simulink model "sfInsectExample"  (R2025b)
settings: Solver=VariableStepAuto  StartTime=0.0  StopTime=24  RelTol=1e-3
PreLoadFcn:
  | load('insect_sim_consts.mat')
  | load('raw_enviro_data.mat')
values from neighbouring files (symbols this model uses):
  cone_angle = 45    [generate_constants.m]
  cone_length = 30    [generate_constants.m]
  fast_vel = 9    [generate_constants.m]
  norm_vel = 6    [generate_constants.m]
  x_bound = [0 100]    [generate_constants.m]
  y_bound = [0 75]    [generate_constants.m]
libraries: simulink_extras x2
settings Model: Creator=The MathWorks, Inc.  LastModifiedBy=The MathWorks, Inc.
settings DataIOCC: ExternalInput=[raw_enviro_data(:,5), raw_enviro_data]  LoadExternalInput=on
settings OptimizationCC: ReuseModelBlockBuffer=off
settings DebuggingCC: UnconnectedInputMsg=warning  UnconnectedOutputMsg=warning  UnconnectedLineMsg=warning
settings ModelReferenceCC: EnableRefExpFcnMdlSchedulingChecks=on
settings RTWCC: GPUComputeCapability=3.5  DLArmComputeVersion=19.05

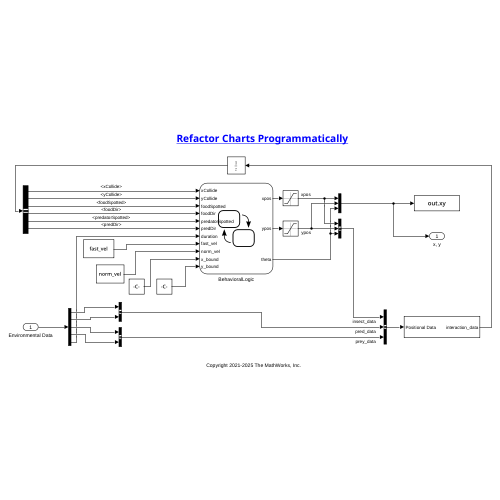
[thumbnail: Simulink's stored preview of the top-level diagram]
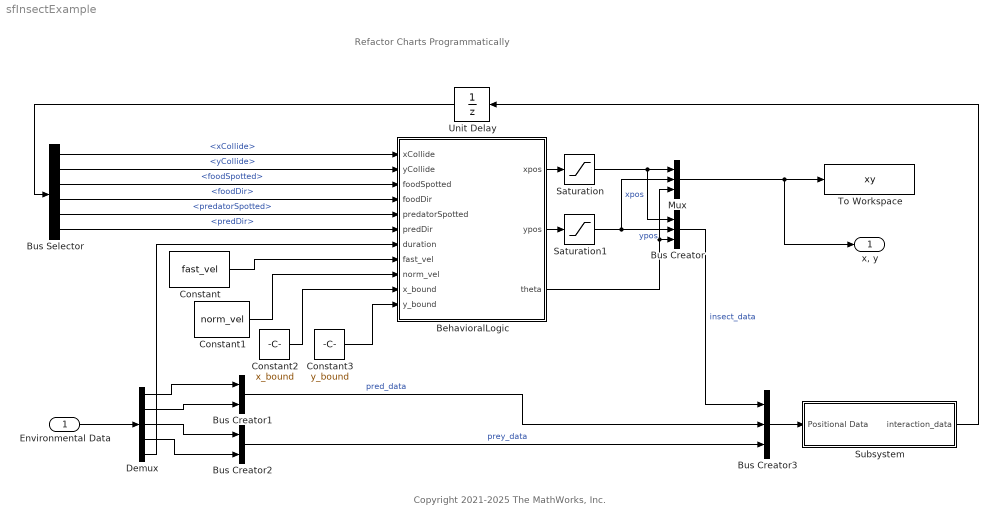
== system sfInsectExample ==
  note: Copyright 2021-2025 The MathWorks, Inc.
  note: Refactor Charts Programmatically
  Environmental Data : Inport
  BehavioralLogic : Stateflow chart  TreatAsAtomicUnit=on
  Bus Creator : BusCreator  Inputs=3
  Bus Creator1 : BusCreator  Inputs=2
  Bus Creator2 : BusCreator  Inputs=2
  Bus Creator3 : BusCreator  Inputs=3
  Bus Selector : BusSelector  OutputSignals=xCollide,yCollide,foodSpotted,foodDir,predatorSpotted,predDir
  Constant : Constant  Value=fast_vel
  Constant1 : Constant  Value=norm_vel
  Constant2 : Constant  Value=x_bound
  Constant3 : Constant  Value=y_bound
  Demux : Demux  Outputs=5
  Mux : Mux  Inputs=3
  Saturation : Saturate  UpperLimit=x_bound(2)  LowerLimit=x_bound(1)
  Saturation1 : Saturate  UpperLimit=y_bound(2)  LowerLimit=y_bound(1)
  Subsystem : Subsystem
  To Workspace : ToWorkspace  VariableName=xy  SampleTime=-1
  Unit Delay : UnitDelay  SampleTime=-1  HasFrameUpgradeWarning=on
  "x, y" : Outport
  wires:
  BehavioralLogic/3(theta) -> Mux/3, Bus Creator/3
  Environmental Data/1 -> Demux/1
  Demux/3 -> Bus Creator2/1
  Demux/4 -> Bus Creator2/2
  Bus Creator3/1 -> Subsystem/1(Positional Data)
  Bus Creator/1 -> Bus Creator3/1  "insect_data"
  Bus Creator1/1 -> Bus Creator3/2  "pred_data"
  Bus Creator2/1 -> Bus Creator3/3  "prey_data"
  Subsystem/1(interaction_data) -> Unit Delay/1
  Bus Selector/1 -> BehavioralLogic/1(xCollide)  "<xCollide>"
  Bus Selector/2 -> BehavioralLogic/2(yCollide)  "<yCollide>"
  Bus Selector/3 -> BehavioralLogic/3(foodSpotted)  "<foodSpotted>"
  Bus Selector/4 -> BehavioralLogic/4(foodDir)  "<foodDir>"
  Bus Selector/5 -> BehavioralLogic/5(predatorSpotted)  "<predatorSpotted>"
  Bus Selector/6 -> BehavioralLogic/6(predDir)  "<predDir>"
  Mux/1 -> To Workspace/1, "x, y"/1
  Demux/1 -> Bus Creator1/1
  Demux/2 -> Bus Creator1/2
  Demux/5 -> BehavioralLogic/7(duration)
  Constant/1 -> BehavioralLogic/8(fast_vel)
  Constant1/1 -> BehavioralLogic/9(norm_vel)
  Unit Delay/1 -> Bus Selector/1
  BehavioralLogic/1(xpos) -> Saturation/1
  Saturation/1 -> Mux/1, Bus Creator/1  "xpos"
  BehavioralLogic/2(ypos) -> Saturation1/1
  Saturation1/1 -> Mux/2, Bus Creator/2  "ypos"
  Constant2/1 -> BehavioralLogic/10(x_bound)
  Constant3/1 -> BehavioralLogic/11(y_bound)

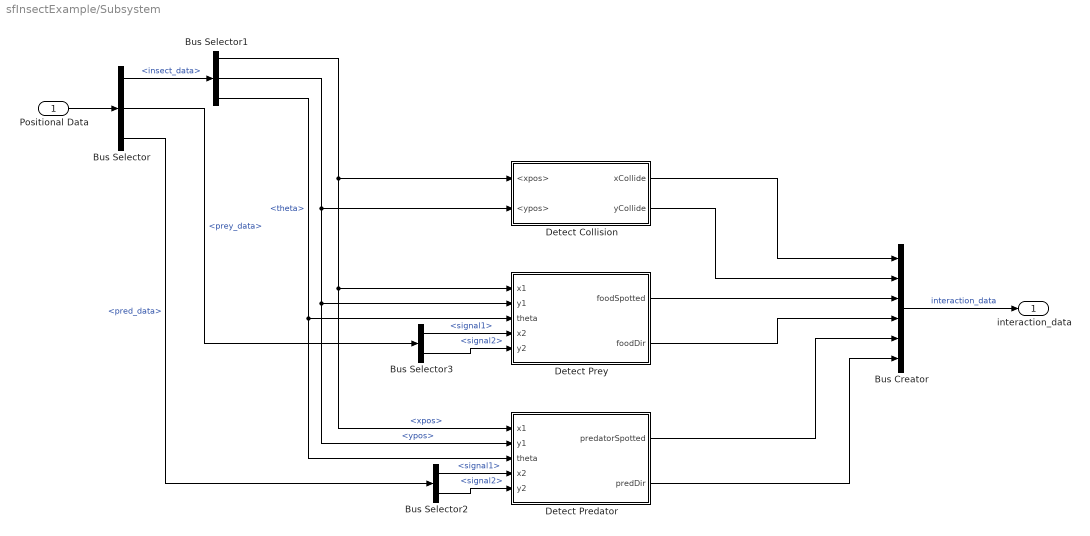
== system sfInsectExample/Subsystem ==
  Positional Data : Inport
  Bus Creator : BusCreator  Inputs=6
  Bus Selector : BusSelector  OutputSignals=insect_data,prey_data,pred_data
  Bus Selector1 : BusSelector  OutputSignals=xpos,ypos,theta
  Bus Selector2 : BusSelector  OutputSignals=signal1,signal2
  Bus Selector3 : BusSelector  OutputSignals=signal1,signal2
  Detect Collision : Subsystem
  "Detect Predator " : Subsystem
  Detect Prey : Subsystem
  interaction_data : Outport
  wires:
  Positional Data/1 -> Bus Selector/1
  Bus Selector/1 -> Bus Selector1/1  "<insect_data>"
  Bus Selector1/1 -> Detect Collision/1(<xpos>), Detect Prey/1(x1), "Detect Predator "/1(x1)  "<xpos>"
  Bus Selector1/2 -> Detect Collision/2(<ypos>), Detect Prey/2(y1), "Detect Predator "/2(y1)  "<ypos>"
  Bus Selector/3 -> Bus Selector2/1  "<pred_data>"
  Bus Selector2/1 -> "Detect Predator "/4(x2)  "<signal1>"
  Bus Selector2/2 -> "Detect Predator "/5(y2)  "<signal2>"
  Bus Selector1/3 -> Detect Prey/3(theta), "Detect Predator "/3(theta)  "<theta>"
  Bus Selector3/1 -> Detect Prey/4(x2)  "<signal1>"
  Bus Selector/2 -> Bus Selector3/1  "<prey_data>"
  Bus Selector3/2 -> Detect Prey/5(y2)  "<signal2>"
  Detect Collision/1(xCollide) -> Bus Creator/1
  Detect Collision/2(yCollide) -> Bus Creator/2
  Detect Prey/1(foodSpotted) -> Bus Creator/3
  Detect Prey/2(foodDir) -> Bus Creator/4
  "Detect Predator "/1(predatorSpotted) -> Bus Creator/5
  "Detect Predator "/2(predDir) -> Bus Creator/6
  Bus Creator/1 -> interaction_data/1  "interaction_data"

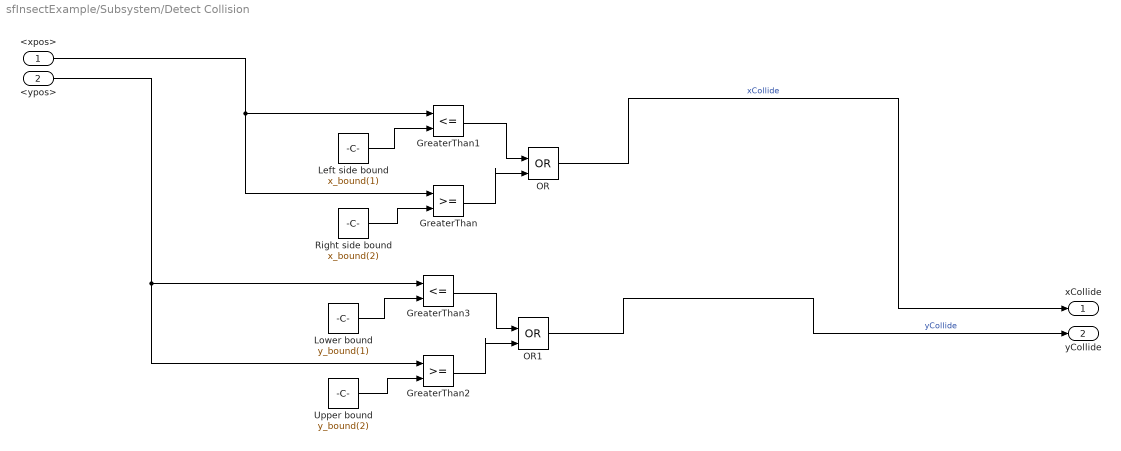
== system sfInsectExample/Subsystem/Detect Collision ==
  <xpos> : Inport
  <ypos> : Inport  Port=2
  GreaterThan : RelationalOperator  OutDataTypeStr=boolean  RndMeth=Simplest  InputSameDT=off
  GreaterThan1 : RelationalOperator  Operator=<=  OutDataTypeStr=boolean  RndMeth=Simplest  InputSameDT=off
  GreaterThan2 : RelationalOperator  OutDataTypeStr=boolean  RndMeth=Simplest  InputSameDT=off
  GreaterThan3 : RelationalOperator  Operator=<=  OutDataTypeStr=boolean  RndMeth=Simplest  InputSameDT=off
  Left side bound : Constant  Value=x_bound(1)
  Lower bound : Constant  Value=y_bound(1)
  OR : Logic  Operator=OR  IconShape=distinctive  AllPortsSameDT=off  OutDataTypeStr=boolean
  OR1 : Logic  Operator=OR  IconShape=distinctive  AllPortsSameDT=off  OutDataTypeStr=boolean
  Right side bound : Constant  Value=x_bound(2)
  Upper bound : Constant  Value=y_bound(2)
  xCollide : Outport
  yCollide : Outport  Port=2
  wires:
  GreaterThan2/1 -> OR1/2
  Upper bound/1 -> GreaterThan2/2
  GreaterThan1/1 -> OR/1
  Right side bound/1 -> GreaterThan/2
  Left side bound/1 -> GreaterThan1/2
  Lower bound/1 -> GreaterThan3/2
  <ypos>/1 -> GreaterThan3/1, GreaterThan2/1
  GreaterThan3/1 -> OR1/1
  <xpos>/1 -> GreaterThan1/1, GreaterThan/1
  GreaterThan/1 -> OR/2
  OR/1 -> xCollide/1  "xCollide"
  OR1/1 -> yCollide/1  "yCollide"

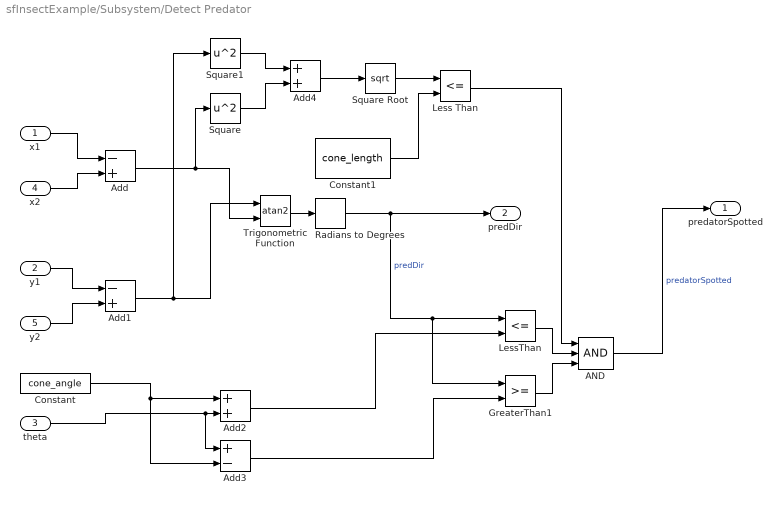
== system sfInsectExample/Subsystem/Detect Predator  ==
  x1 : Inport
  y1 : Inport  Port=2
  theta : Inport  Port=3
  x2 : Inport  Port=4
  y2 : Inport  Port=5
  AND : Logic  Inputs=3  IconShape=distinctive  AllPortsSameDT=off  OutDataTypeStr=boolean
  Add : Sum  Inputs=-+
  Add1 : Sum  Inputs=-+
  Add2 : Sum
  Add3 : Sum  Inputs=+-
  Add4 : Sum
  Constant : Constant  Value=cone_angle
  Constant1 : Constant  Value=cone_length
  GreaterThan1 : RelationalOperator  OutDataTypeStr=boolean  RndMeth=Simplest  InputSameDT=off
  Less Than : RelationalOperator  Operator=<=  OutDataTypeStr=boolean  RndMeth=Simplest  InputSameDT=off
  LessThan : RelationalOperator  Operator=<=  OutDataTypeStr=boolean  RndMeth=Simplest  InputSameDT=off
  Radians to Degrees : simulink_extras/Transformations/Radians to Degrees
  Square : Math  Operator=square
  Square Root : Sqrt
  Square1 : Math  Operator=square
  Trigonometric Function : Trigonometry  Operator=atan2
  predatorSpotted : Outport
  predDir : Outport  Port=2
  wires:
  x1/1 -> Add/1
  x2/1 -> Add/2
  y1/1 -> Add1/1
  y2/1 -> Add1/2
  Add1/1 -> Trigonometric Function/1, Square1/1
  Add/1 -> Square/1, Trigonometric Function/2
  Trigonometric Function/1 -> Radians to Degrees/1
  Radians to Degrees/1 -> predDir/1, GreaterThan1/1, LessThan/1  "predDir"
  theta/1 -> Add3/1, Add2/2
  Constant/1 -> Add3/2, Add2/1
  Add2/1 -> LessThan/2
  Add3/1 -> GreaterThan1/2
  LessThan/1 -> AND/2
  GreaterThan1/1 -> AND/3
  Square1/1 -> Add4/1
  Square/1 -> Add4/2
  Add4/1 -> Square Root/1
  Square Root/1 -> Less Than/1
  Constant1/1 -> Less Than/2
  Less Than/1 -> AND/1
  AND/1 -> predatorSpotted/1  "predatorSpotted"

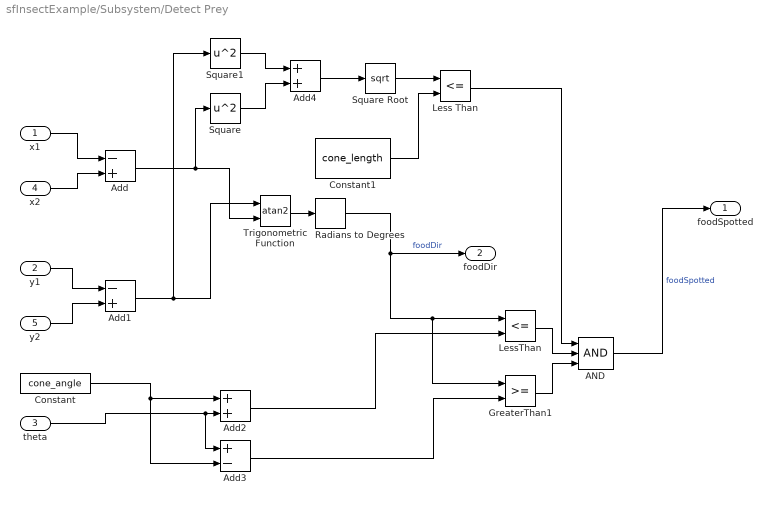
== system sfInsectExample/Subsystem/Detect Prey ==
  x1 : Inport
  y1 : Inport  Port=2
  theta : Inport  Port=3
  x2 : Inport  Port=4
  y2 : Inport  Port=5
  AND : Logic  Inputs=3  IconShape=distinctive  AllPortsSameDT=off  OutDataTypeStr=boolean
  Add : Sum  Inputs=-+
  Add1 : Sum  Inputs=-+
  Add2 : Sum
  Add3 : Sum  Inputs=+-
  Add4 : Sum
  Constant : Constant  Value=cone_angle
  Constant1 : Constant  Value=cone_length
  GreaterThan1 : RelationalOperator  OutDataTypeStr=boolean  RndMeth=Simplest  InputSameDT=off
  Less Than : RelationalOperator  Operator=<=  OutDataTypeStr=boolean  RndMeth=Simplest  InputSameDT=off
  LessThan : RelationalOperator  Operator=<=  OutDataTypeStr=boolean  RndMeth=Simplest  InputSameDT=off
  Radians to Degrees : simulink_extras/Transformations/Radians to Degrees
  Square : Math  Operator=square
  Square Root : Sqrt
  Square1 : Math  Operator=square
  Trigonometric Function : Trigonometry  Operator=atan2
  foodSpotted : Outport
  foodDir : Outport  Port=2
  wires:
  x1/1 -> Add/1
  x2/1 -> Add/2
  y1/1 -> Add1/1
  y2/1 -> Add1/2
  Add1/1 -> Trigonometric Function/1, Square1/1
  Add/1 -> Square/1, Trigonometric Function/2
  Trigonometric Function/1 -> Radians to Degrees/1
  Radians to Degrees/1 -> foodDir/1, GreaterThan1/1, LessThan/1  "foodDir"
  theta/1 -> Add3/1, Add2/2
  Constant/1 -> Add3/2, Add2/1
  Add2/1 -> LessThan/2
  Add3/1 -> GreaterThan1/2
  LessThan/1 -> AND/2
  GreaterThan1/1 -> AND/3
  Square1/1 -> Add4/1
  Square/1 -> Add4/2
  Add4/1 -> Square Root/1
  Square Root/1 -> Less Than/1
  Constant1/1 -> Less Than/2
  Less Than/1 -> AND/1
  AND/1 -> foodSpotted/1  "foodSpotted"

== stateflow chart sfInsectExample/BehavioralLogic ==
  state Awake
    xpos = xpos + vel*cos(deg2rad(theta));
    ypos = ypos + vel*sin(deg2rad(theta));
    state Safe
      flee_time = 0;
      state searching
        state normal
        state xBump
          theta = 180-theta;
          xpos = min(x_bound(2),max(xpos,x_bound(1)));
        state yBump
          theta = -1*theta;
          ypos = min(y_bound(2),max(ypos,y_bound(1)));
        (default) -> normal
        normal -> Awake.Safe.searching.xBump [order 2] : [xCollide]
        normal -> Awake.Safe.searching.yBump [order 1] : [yCollide]
        Awake.Safe.searching.xBump -> normal
        Awake.Safe.searching.yBump -> normal
      state Hunting
      (default) -> searching
      searching -> Hunting : [foodSpotted]{vel=fast_vel;theta=foodDir;}
      Hunting -> searching : [foodSpotted == false]{vel=norm_vel;}
    state Danger
      flee_time = flee_time+1;
      state Normal
        entry, during:
        theta = predDir + 180;
      state xBump
        theta = 180-theta;
        xpos = min(x_bound(2),max(xpos,x_bound(1)));
      state yBump
        theta = -1*theta;
        ypos = min(y_bound(2),max(ypos,y_bound(1)));
      (default) -> Normal
      (junction 161) -> (junction 135)
      Normal -> (junction 161) [order 2]
      Normal -> (junction 163) [order 1]
      (junction 163) -> (junction 141)
      (junction 135) -> (junction 153) : [xCollide]
      (junction 141) -> (junction 155) : [yCollide]
      (junction 143) -> Normal
      (junction 147) -> (junction 143)
      (junction 138) -> (junction 143)
      (junction 153) -> Awake.Danger.xBump
      Awake.Danger.xBump -> (junction 147)
      Awake.Danger.yBump -> (junction 138)
      (junction 155) -> Awake.Danger.yBump
    (default) -> Safe
    Safe -> Danger : [predatorSpotted]{vel = fast_vel;}
    Danger -> Safe : [predatorSpotted == 0 & flee_time >= 3]{vel=norm_vel;}
  state Asleep
  (default) -> Awake
  Awake -> Asleep : [duration >= 12]
  Asleep -> Awake : [duration >= 24]
  data: xCollide input; yCollide input; foodSpotted input; foodDir input; vel local =norm_vel; predatorSpotted input; xpos output =1; ypos output =1; predDir input; duration input; theta output =randi(90); fast_vel input; norm_vel input; x_bound input; y_bound input; flee_time local
